simulink model "eesm_corroboration"  (R2026a)
settings: Solver=ode3  StopTime=1.5  FixedStep=Ts_eesm
undefined symbols (not defined in the file or in its folder): Id_ref, If_ref, Iq_ref, J_kgm2, pole_pairs, rpm_grid, Status_tbl, t_grid, tau_f_s, tau_s_s
settings Model: Creator=darsh  LastModifiedBy=darsh

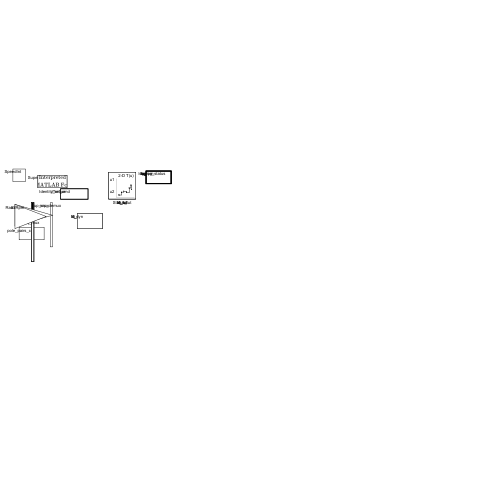
[thumbnail: Simulink's stored preview of the top-level diagram]
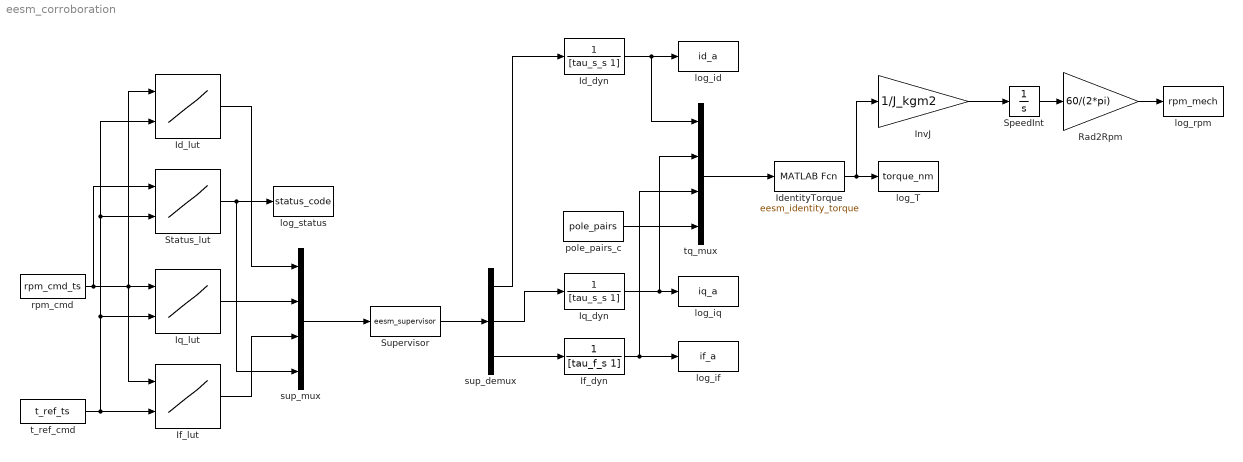
== system eesm_corroboration ==
  Id_dyn : TransferFcn  Denominator=[tau_s_s 1]
  Id_lut : Lookup_n-D  BreakpointsForDimension1=rpm_grid  BreakpointsForDimension2=t_grid  BreakpointsForDimension3=[5, 7]  Table=Id_ref  ExtrapMethod=Clip  InternalRulePriority=Speed  RndMeth=Simplest
      settings: InputPortMap=u0,u1
  IdentityTorque : MATLABFcn  MATLABFcn=eesm_identity_torque
  If_dyn : TransferFcn  Denominator=[tau_f_s 1]
  If_lut : Lookup_n-D  BreakpointsForDimension1=rpm_grid  BreakpointsForDimension2=t_grid  BreakpointsForDimension3=[5, 7]  Table=If_ref  ExtrapMethod=Clip  InternalRulePriority=Speed  RndMeth=Simplest
      settings: InputPortMap=u0,u1
  InvJ : Gain  Gain=1/J_kgm2
  Iq_dyn : TransferFcn  Denominator=[tau_s_s 1]
  Iq_lut : Lookup_n-D  BreakpointsForDimension1=rpm_grid  BreakpointsForDimension2=t_grid  BreakpointsForDimension3=[5, 7]  Table=Iq_ref  ExtrapMethod=Clip  InternalRulePriority=Speed  RndMeth=Simplest
      settings: InputPortMap=u0,u1
  Rad2Rpm : Gain  Gain=60/(2*pi)
  SpeedInt : Integrator
  Status_lut : Lookup_n-D  BreakpointsForDimension1=rpm_grid  BreakpointsForDimension2=t_grid  BreakpointsForDimension3=[5, 7]  Table=Status_tbl  InterpMethod=Nearest  ExtrapMethod=Clip  InternalRulePriority=Speed  RndMeth=Simplest
      settings: InputPortMap=u0,u1
  Supervisor : MATLABFcn  MATLABFcn=eesm_supervisor
  log_T : ToWorkspace  VariableName=torque_nm  SaveFormat=Timeseries  SampleTime=-1
  log_id : ToWorkspace  VariableName=id_a  SaveFormat=Timeseries  SampleTime=-1
  log_if : ToWorkspace  VariableName=if_a  SaveFormat=Timeseries  SampleTime=-1
  log_iq : ToWorkspace  VariableName=iq_a  SaveFormat=Timeseries  SampleTime=-1
  log_rpm : ToWorkspace  VariableName=rpm_mech  SaveFormat=Timeseries  SampleTime=-1
  log_status : ToWorkspace  VariableName=status_code  SaveFormat=Timeseries  SampleTime=-1
  pole_pairs_c : Constant  Value=pole_pairs
  rpm_cmd : FromWorkspace  VariableName=rpm_cmd_ts
  sup_demux : Demux  Outputs=3
  sup_mux : Mux
  t_ref_cmd : FromWorkspace  VariableName=t_ref_ts
  tq_mux : Mux
  wires:
  rpm_cmd/1 -> Id_lut/1, Iq_lut/1, If_lut/1, Status_lut/1
  t_ref_cmd/1 -> Id_lut/2, Status_lut/2, Iq_lut/2, If_lut/2
  Supervisor/1 -> sup_demux/1
  Id_lut/1 -> sup_mux/1
  Iq_lut/1 -> sup_mux/2
  sup_mux/1 -> Supervisor/1
  Status_lut/1 -> sup_mux/4, log_status/1
  If_lut/1 -> sup_mux/3
  sup_demux/1 -> Id_dyn/1
  sup_demux/2 -> Iq_dyn/1
  sup_demux/3 -> If_dyn/1
  Id_dyn/1 -> tq_mux/1, log_id/1
  pole_pairs_c/1 -> tq_mux/4
  Iq_dyn/1 -> tq_mux/2, log_iq/1
  tq_mux/1 -> IdentityTorque/1
  If_dyn/1 -> tq_mux/3, log_if/1
  InvJ/1 -> SpeedInt/1
  IdentityTorque/1 -> InvJ/1, log_T/1
  SpeedInt/1 -> Rad2Rpm/1
  Rad2Rpm/1 -> log_rpm/1
